simulink model "Semi Converter"  (R2025a)
settings: Solver=VariableStepAuto  StartTime=0.0  StopTime=5.0  RelTol=1e-3
libraries: spsDiodeLib x2, spsMultimeterLib x2, spsThyristorLib x2, spsACVoltageSourceLib x1, spsSeriesRLCBranchLib x1, sps_lib x1
settings Model: Creator=Ayush  LastModifiedBy=Ayush

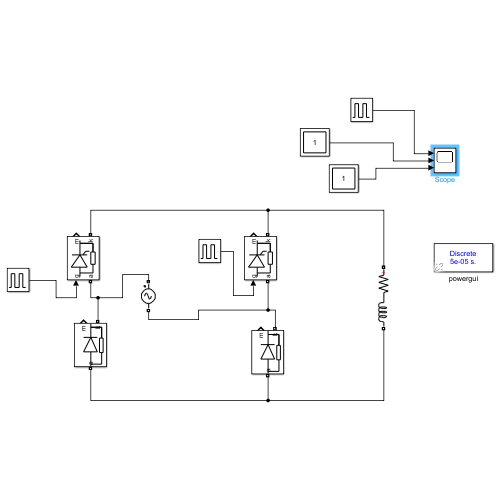
[thumbnail: Simulink's stored preview of the top-level diagram]
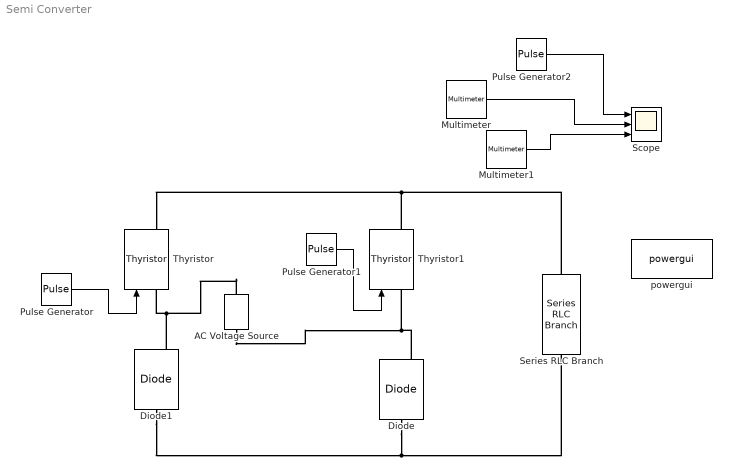
== system Semi Converter ==
  AC Voltage Source : spsACVoltageSourceLib/AC Voltage Source  Amplitude=325.27  Phase=0  Frequency=50  SampleTime=0  Measurements=None  BusType=swing  Pref=10e3  Qref=0  Qmin=-inf  Qmax=+inf
  Diode : spsDiodeLib/Diode  Ron=0.001  Lon=0  Vf=0.8  IC=0  UseSnubber=0  Rs=500  Cs=250e-9  Measurements=on
  Diode1 : spsDiodeLib/Diode  Ron=0.001  Lon=0  Vf=0.8  IC=0  UseSnubber=0  Rs=500  Cs=250e-9  Measurements=on
  Multimeter : spsMultimeterLib/Multimeter  L=2  sel=1  yselected={}  Gain=1  OutputType=Complex  PlotAtSimulationStop=off  PhasorSimulation=off
  Multimeter1 : spsMultimeterLib/Multimeter  L=2  sel=2  yselected={}  Gain=1  OutputType=Complex  PlotAtSimulationStop=off  PhasorSimulation=off
  Pulse Generator : DiscretePulseGenerator  PulseType=Time based  Period=0.02  PulseWidth=5  PhaseDelay=0.00167  VectorParams1D=off
  Pulse Generator1 : DiscretePulseGenerator  PulseType=Time based  Period=0.02  PulseWidth=5  PhaseDelay=0.01167  VectorParams1D=off
  Pulse Generator2 : DiscretePulseGenerator  PulseType=Time based  Period=0.01  PulseWidth=5  PhaseDelay=0.0016
  Scope : Scope  NumInputPorts=3
      settings: ActiveDisplayString=3  ActiveDisplayYMinimum=-1.5885951750146381  ActiveDisplayYMaximum=19.219906753450207
  Series RLC Branch : spsSeriesRLCBranchLib/Series RLC Branch  LConnTagsString=__new0  RConnTagsString=__new0  BranchType=RL  Resistance=20  Inductance=0.03  SetiL0=off  InitialCurrent=0  Capacitance=1e-6  Setx0=off  InitialVoltage=0  Measurements=Branch voltage and current
  Thyristor : spsThyristorLib/Thyristor  Ron=0.001  Lon=0  Vf=0.8  IC=0  Rs=500  Cs=250e-9  Measurements=on
  Thyristor1 : spsThyristorLib/Thyristor  Ron=0.001  Lon=0  Vf=0.8  IC=0  Rs=500  Cs=250e-9  Measurements=on
  powergui : sps_lib/powergui  Priority=1  SimulationMode=Discrete  SampleTime=50e-6  frequency=60  Iterations=50  frequencyindice=50  Pbase=100e6  ErrMax=1e-4  UnitsV=kV  UnitsW=MW  buscounter=0  FunctionMessages=off  echomessages=off  EnableUseOfTLC=off  CurrentSourceSwitches=off  DisableSnubberDevices=off  DisableRonSwitches=off  DisableVfSwitches=off  DisplayEquations=off  AutomaticDiscreteSolvers=off  SolverType=Tustin/Backward Euler (TBE)  Interpol=off  ExternalGateDelay=off  methode=off  Ts=100  x0status=blocks  SPID=on  SwTol=0  HookPort=off  NonlinearTolerance=1e-4  nMaxIteration=100  ContinueOnMaxIteration=off  RestoreLinks=warning  ResistiveCurrentMeasurement=off  Frange=[0:2:500]  Ylog=off  Xlog=on  ShowGrid=off  save=off  variable=ZData  structure=0  ZoomFFT=off  StartTime=0.0  cycles=1  DisplayStyle=1  fundamental=60  FreqAxis=off  MaxFrequency=1000  frequencyindicesteady=1  RmsSteady=1  display=off
  wires:
  Pulse Generator/1 -> Thyristor/1
  Pulse Generator1/1 -> Thyristor1/1
  Multimeter/1 -> Scope/2
  Multimeter1/1 -> Scope/3
  Pulse Generator2/1 -> Scope/1
  connections:
  AC Voltage Source/RConn1 -- Thyristor/LConn1 -- Diode1/RConn1
  Thyristor1/RConn1 -- Series RLC Branch/LConn1 -- Thyristor/RConn1
  AC Voltage Source/LConn1 -- Diode/RConn1 -- Thyristor1/LConn1
  Series RLC Branch/RConn1 -- Diode1/LConn1 -- Diode/LConn1
